simulink model "Cable_Wo_M_Inductance_Modelling_Study"  (R2024b)
settings: Solver=FixedStepDiscrete  StartTime=0.0  StopTime=5  FixedStep=1e-6  RelTol=1e-3  AbsTol=1
values from neighbouring files (symbols this model uses):
  Ccs1 = 733.62e-12    (= 7.3362e-10)    [Cable_Data_Inductance_Study.m]
  Ccs2 = 733.62e-12    (= 7.3362e-10)    [Cable_Data_Inductance_Study.m]
  Lc1 = 0.092e-6    (= 9.2e-08)    [Cable_Data_Inductance_Study.m]
  Lc1_total = Lc1 + Mcs1    (= 2.72e-07)    [Cable_Data_Inductance_Study.m]
  Lc2 = 0.092e-6    (= 9.2e-08)    [Cable_Data_Inductance_Study.m]
  Lc2_total = Lc2 + Mcs2    (= 2.72e-07)    [Cable_Data_Inductance_Study.m]
  Len35_batt1_HVJB1_neg = 0.600    (= 0.6)    [Cable_Data_Inductance_Study.m]
  Len35_batt1_HVJB1_pos = 0.750    (= 0.75)    [Cable_Data_Inductance_Study.m]
  Ls1_eff = Ls1 + Mss_cal    [Cable_Data_Inductance_Study.m]
  Ls2_eff = Ls2 + Mss_cal    [Cable_Data_Inductance_Study.m]
  Rc1 = 0.38e-3    (= 0.00038)    [Cable_Data_Inductance_Study.m]
  Rc2 = 0.38e-3    (= 0.00038)    [Cable_Data_Inductance_Study.m]
  Rs1 = 2.55e-3    (= 0.00255)    [Cable_Data_Inductance_Study.m]
  Rs2 = 2.55e-3    (= 0.00255)    [Cable_Data_Inductance_Study.m]
undefined symbols (not defined in the file or in its folder): DiscIntNeverNeededParam, Lns95, Lps95
libraries: spsSeriesRLCBranchLib x59, spsCurrentMeasurementLib x12, spsVoltageMeasurementLib x9, spsGroundLib x6, spsMultimeterLib x6, eeGeneralControl x2, spsVariableResistorLib x2, spsDCVoltageSourceLib x2, spspowerguiLib x1, sps_lib x1
(part 1 of 2)
settings Model: Creator=SUDHAK1  LastModifiedBy=SUDHAK1

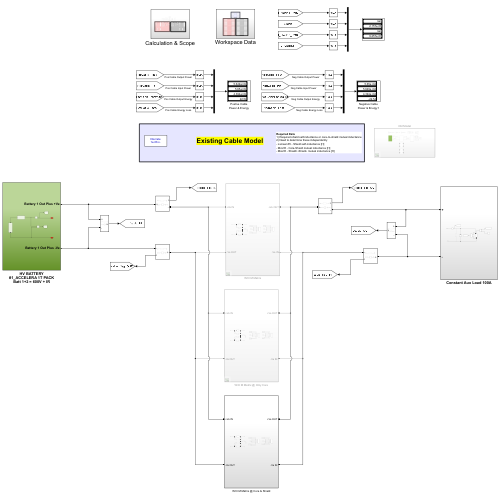
[thumbnail: Simulink's stored preview of the top-level diagram]
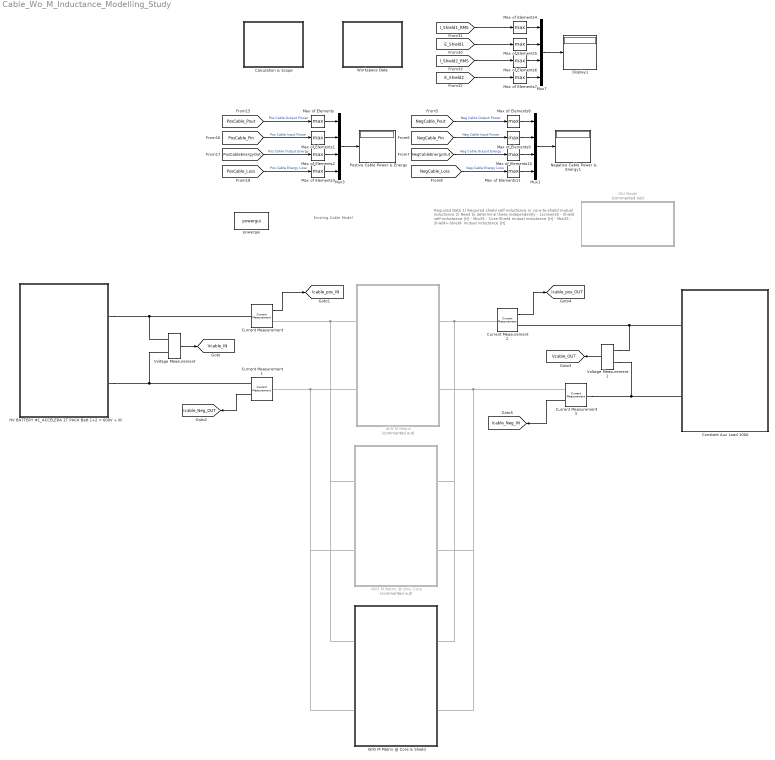
== system Cable_Wo_M_Inductance_Modelling_Study ==
  note: Required Data
      | 1) Required shield self-inductance or core-to-shield mutual inductance
      | 2) Need to determine these independently
      | - Lscreen35 - Shield self-inductance [H]
      | - Mcs35 - Core-Shield mutual inductance [H]
      | - Mss35 - Shield+-Shield- mutual inductance [H]
  note: Existing Cable Model
  Calculation & Scope : Subsystem
  Constant Aux Load 100A : Subsystem
  Current Measurement{,1..3} (4 alike) : spsCurrentMeasurementLib/Current Measurement  PhasorSimulation=off  OutputType=Complex  PSBequivalent=0
  Display1 : Display
  HV BATTERY #1_ACCELERA 1T PACK Batt 1+2 = 600V + IR : Subsystem
  Max of Elements{,1..11} (12 alike) : MinMax  Function=max
  Mux1 : Mux
  Mux3 : Mux
  Mux7 : Mux
  Negative Cable Power & Energy1 : Display
  Old Model : Subsystem  Commented=on
  Postive Cable Power & Energy : Display
  Voltage Measurement : spsVoltageMeasurementLib/Voltage Measurement  PhasorSimulation=off  OutputType=Complex  PSBequivalent=0
  Voltage Measurement1 : spsVoltageMeasurementLib/Voltage Measurement  PhasorSimulation=off  OutputType=Complex  PSBequivalent=0
  W/O M Matrix : Subsystem  Commented=on
  W/O M Matrix @ Core & Shield : Subsystem
  W/O M Matrix @ Only Core : Subsystem  Commented=on
  Workspace Data : Subsystem
  powergui : sps_lib/powergui  Priority=1  SimulationMode=Discrete  SampleTime=1e-6  frequency=60  Iterations=50  frequencyindice=0  Pbase=100e6  ErrMax=1e-4  UnitsV=kV  UnitsW=MW  buscounter=0  FunctionMessages=off  echomessages=off  EnableUseOfTLC=off  CurrentSourceSwitches=off  DisableSnubberDevices=off  DisableRonSwitches=off  DisableVfSwitches=off  DisplayEquations=off  AutomaticDiscreteSolvers=off  SolverType=Tustin/Backward Euler (TBE)  Interpol=off  ExternalGateDelay=off  methode=off  Ts=100  x0status=blocks  SPID=on  SwTol=0  HookPort=off  NonlinearTolerance=1e-4  nMaxIteration=100  ContinueOnMaxIteration=off  RestoreLinks=warning  ResistiveCurrentMeasurement=off  Frange=[0:2:500]  Ylog=off  Xlog=on  ShowGrid=off  save=off  variable=ZData  structure=0  ZoomFFT=off  StartTime=0.0  cycles=1  DisplayStyle=1  fundamental=60  FreqAxis=off  MaxFrequency=1000  frequencyindicesteady=1  RmsSteady=1  display=off
  tag scope: Icable_Neg_IN=global, Icable_Neg_OUT=global, Icable_pos_IN=global, Icable_pos_OUT=global, Vcable_IN=global, Vcable_OUT=global
  wires:
  Voltage Measurement1/1 -> [Vcable_OUT]
  Voltage Measurement/1 -> [Vcable_IN]
  Current Measurement/1 -> [Icable_pos_IN]
  Current Measurement3/1 -> [Icable_Neg_IN]
  Current Measurement1/1 -> [Icable_Neg_OUT]
  Current Measurement2/1 -> [Icable_pos_OUT]
  Max of Elements8/1 -> Mux1/1
  Mux1/1 -> Negative Cable Power & Energy1/1
  Max of Elements9/1 -> Mux1/2
  Max of Elements10/1 -> Mux1/3
  [PosCable_Pout] -> Max of Elements/1  "Pos Cable Output Power"
  Max of Elements11/1 -> Mux1/4
  [NegCableEnergyOut] -> Max of Elements10/1  "Neg Cable Output Energy"
  [PosCable_Pin] -> Max of Elements1/1  "Pos Cable Input Power"
  [E_Shield2] -> Max of Elements7/1
  Max of Elements7/1 -> Mux7/4
  Max of Elements5/1 -> Mux7/2
  [I_Shield2_RMS] -> Max of Elements6/1
  Max of Elements4/1 -> Mux7/1
  Max of Elements6/1 -> Mux7/3
  Mux7/1 -> Display1/1
  [E_Shield1] -> Max of Elements5/1
  [PosCableEnergyOut] -> Max of Elements2/1  "Pos Cable Output Energy"
  Max of Elements3/1 -> Mux3/4
  [I_Shield1_RMS] -> Max of Elements4/1
  [PosCable_Loss] -> Max of Elements3/1  "Pos Cable Energy Loss"
  Max of Elements2/1 -> Mux3/3
  [NegCable_Pin] -> Max of Elements9/1  "Neg Cable Input Power"
  Max of Elements/1 -> Mux3/1
  [NegCable_Loss] -> Max of Elements11/1  "Neg Cable Energy Loss"
  Max of Elements1/1 -> Mux3/2
  Mux3/1 -> Postive Cable Power & Energy/1
  [NegCable_Pout] -> Max of Elements8/1  "Neg Cable Output Power"
  connections:
  Voltage Measurement/LConn2 -- HV BATTERY #1_ACCELERA 1T PACK Batt 1+2 = 600V + IR/RConn2 -- Current Measurement1/RConn1
  Constant Aux Load 100A/RConn1 -- Voltage Measurement1/LConn1 -- Current Measurement2/RConn1
  Voltage Measurement1/LConn2 -- Constant Aux Load 100A/RConn2 -- Current Measurement3/LConn1
  HV BATTERY #1_ACCELERA 1T PACK Batt 1+2 = 600V + IR/RConn1 -- Voltage Measurement/LConn1 -- Current Measurement/LConn1
  W/O M Matrix/LConn1 -- W/O M Matrix @ Core & Shield/LConn1 -- W/O M Matrix @ Only Core/LConn1 -- Current Measurement/RConn1
  W/O M Matrix/RConn1 -- W/O M Matrix @ Core & Shield/RConn1 -- W/O M Matrix @ Only Core/RConn1 -- Current Measurement2/LConn1
  W/O M Matrix/LConn2 -- W/O M Matrix @ Core & Shield/LConn2 -- W/O M Matrix @ Only Core/LConn2 -- Current Measurement1/LConn1
  W/O M Matrix/RConn2 -- W/O M Matrix @ Core & Shield/RConn2 -- W/O M Matrix @ Only Core/RConn2 -- Current Measurement3/RConn1

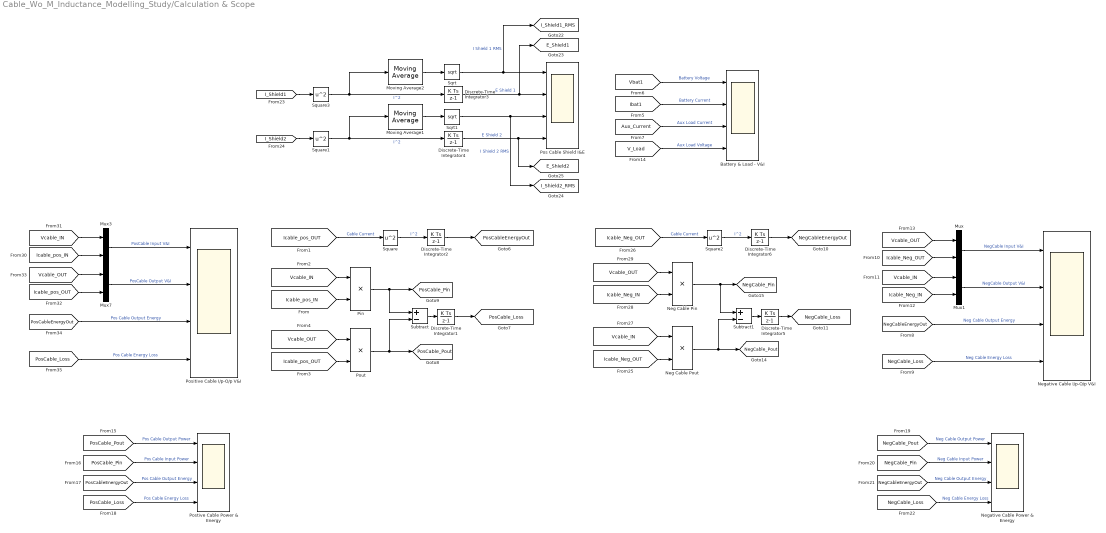
== system Cable_Wo_M_Inductance_Modelling_Study/Calculation & Scope ==
  Battery & Load - V&I : Scope  NumInputPorts=4
  Discrete-Time Integrator{1..6} (6 alike) : DiscreteIntegrator  SampleTime=-1  ICPrevOutput=DiscIntNeverNeededParam  ICPrevScaledInput=DiscIntNeverNeededParam
  Moving Average1 : eeGeneralControl/Moving Average  VariantControl=Variant1  LabelModeActiveChoice=Discrete  f=60  x0=0  BufferSize=8192  Ts=-1
  Moving Average2 : eeGeneralControl/Moving Average  VariantControl=Variant1  LabelModeActiveChoice=Discrete  f=60  x0=0  BufferSize=8192  Ts=-1
  Mux{,1,3,7} (4 alike) : Mux  Inputs=2
  Neg Cable Pin : Product
  Neg Cable Pout : Product
  Negative Cable Power & Energy : Scope  NumInputPorts=4
  Negative Cable I/p-O/p V&I : Scope  NumInputPorts=4
  Pin : Product
  Pos Cable Shield I&E : Scope  NumInputPorts=4
  Positive Cable I/p-O/p V&I : Scope  NumInputPorts=4
  Postive Cable Power & Energy : Scope  NumInputPorts=4
  Pout : Product
  Sqrt : Sqrt
  Sqrt1 : Sqrt
  Square{,1..3} (4 alike) : Math  Operator=square
  Subtract : Sum  Inputs=+-
  Subtract1 : Sum  Inputs=+-
  tag scope: E_Shield1=global, E_Shield2=global, I_Shield1_RMS=global, I_Shield2_RMS=global, NegCableEnergyOut=global, NegCable_Loss=global, NegCable_Pin=global, NegCable_Pout=global, PosCableEnergyOut=global, PosCable_Loss=global, PosCable_Pin=global, PosCable_Pout=global
  wires:
  [NegCableEnergyOut] -> Negative Cable I/p-O/p V&I/3  "Neg Cable Output Energy"
  Moving Average2/1 -> Sqrt/1
  Square/1 -> Discrete-Time Integrator2/1  "I^2"
  [Icable_pos_IN] -> Pin/2
  [PosCableEnergyOut] -> Postive Cable Power & Energy/3  "Pos Cable Output Energy"
  [Icable_pos_OUT] -> Pout/2
  [Icable_pos_OUT] -> Square/1  "Cable Current"
  Moving Average1/1 -> Sqrt1/1
  Discrete-Time Integrator3/1 -> [E_Shield1], Pos Cable Shield I&E/2  "E Shield 1"
  Pin/1 -> [PosCable_Pin], Subtract/1
  [Vcable_OUT] -> Pout/1
  Mux/1 -> Negative Cable I/p-O/p V&I/1  "NegCable Input V&I"
  [Aux_Current] -> Battery & Load - V&I/3  "Aux Load Current"
  [V_Load] -> Battery & Load - V&I/4  "Aux Load Voltage"
  [Icable_Neg_OUT] -> Mux/2
  Discrete-Time Integrator4/1 -> Pos Cable Shield I&E/4, [E_Shield2]  "E Shield 2"
  Square3/1 -> Discrete-Time Integrator3/1, Moving Average2/1  "I^2"
  [I_Shield1] -> Square3/1
  [Vbat1] -> Battery & Load - V&I/1  "Battery Voltage"
  Discrete-Time Integrator1/1 -> [PosCable_Loss]
  Sqrt1/1 -> Pos Cable Shield I&E/3, [I_Shield2_RMS]  "I Shield 2 RMS"
  [Vcable_IN] -> Neg Cable Pout/1
  [NegCable_Loss] -> Negative Cable I/p-O/p V&I/4  "Neg Cable Energy Loss"
  Subtract/1 -> Discrete-Time Integrator1/1
  Pout/1 -> Subtract/2, [PosCable_Pout]
  [Icable_Neg_OUT] -> Square2/1  "Cable Current"
  [PosCable_Pin] -> Postive Cable Power & Energy/2  "Pos Cable Input Power"
  [I_Shield2] -> Square1/1
  Mux1/1 -> Negative Cable I/p-O/p V&I/2  "NegCable Output V&I"
  Discrete-Time Integrator2/1 -> [PosCableEnergyOut]
  [Vcable_IN] -> Pin/1
  Square1/1 -> Discrete-Time Integrator4/1, Moving Average1/1  "I^2"
  [Icable_Neg_IN] -> Mux1/2
  [PosCable_Pout] -> Postive Cable Power & Energy/1  "Pos Cable Output Power"
  [PosCable_Loss] -> Postive Cable Power & Energy/4  "Pos Cable Energy Loss"
  [Ibat1] -> Battery & Load - V&I/2  "Battery Current"
  Sqrt/1 -> Pos Cable Shield I&E/1, [I_Shield1_RMS]  "I Shield 1 RMS"
  Subtract1/1 -> Discrete-Time Integrator5/1
  Discrete-Time Integrator5/1 -> [NegCable_Loss]
  Neg Cable Pout/1 -> Subtract1/2, [NegCable_Pout]
  Discrete-Time Integrator6/1 -> [NegCableEnergyOut]
  [Vcable_OUT] -> Neg Cable Pin/1
  Neg Cable Pin/1 -> Subtract1/1, [NegCable_Pin]
  [Icable_Neg_IN] -> Neg Cable Pin/2
  [Icable_Neg_OUT] -> Neg Cable Pout/2
  Square2/1 -> Discrete-Time Integrator6/1  "I^2"
  [NegCable_Loss] -> Negative Cable Power & Energy/4  "Neg Cable Energy Loss"
  [NegCableEnergyOut] -> Negative Cable Power & Energy/3  "Neg Cable Output Energy"
  [NegCable_Pout] -> Negative Cable Power & Energy/1  "Neg Cable Output Power"
  [NegCable_Pin] -> Negative Cable Power & Energy/2  "Neg Cable Input Power"
  [Icable_pos_IN] -> Mux3/2
  [Vcable_IN] -> Mux3/1
  [Icable_pos_OUT] -> Mux7/2
  [PosCable_Loss] -> Positive Cable I/p-O/p V&I/4  "Pos Cable Energy Loss"
  Mux3/1 -> Positive Cable I/p-O/p V&I/1  "PosCable Input V&I"
  Mux7/1 -> Positive Cable I/p-O/p V&I/2  "PosCable Output V&I"
  [Vcable_OUT] -> Mux7/1
  [PosCableEnergyOut] -> Positive Cable I/p-O/p V&I/3  "Pos Cable Output Energy"
  [Vcable_IN] -> Mux1/1
  [Vcable_OUT] -> Mux/1

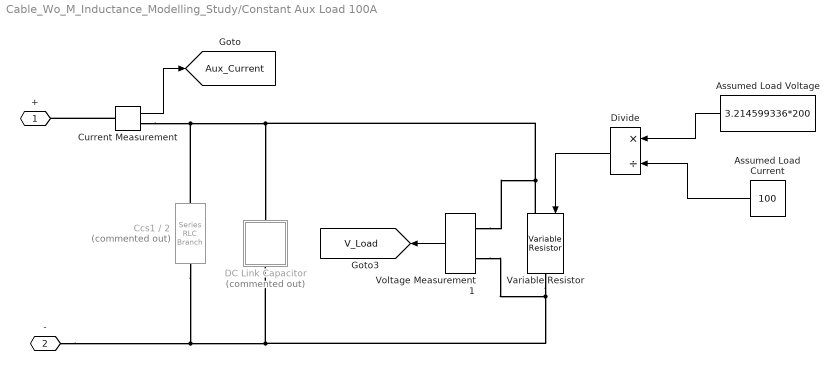
== system Cable_Wo_M_Inductance_Modelling_Study/Constant Aux Load 100A ==
  " Ccs1 / 2" : spsSeriesRLCBranchLib/Series RLC Branch  Commented=on  LConnTagsString=__new0  RConnTagsString=__new0  BranchType=R  Resistance=1  Inductance=1e-3  SetiL0=off  InitialCurrent=0  Capacitance=Ccs1/2  Setx0=off  InitialVoltage=0  Measurements=None
  Assumed Load Current : Constant  Value=100
  Assumed Load Voltage : Constant  Value=3.214599336*200
  Current Measurement : spsCurrentMeasurementLib/Current Measurement  PhasorSimulation=off  OutputType=Complex  PSBequivalent=0
  DC Link Capacitor : Subsystem  Commented=on
      settings: PortSchema="{\"entries\":[{\"content\":{\"sides\":[{\"content\":{},\"type\":\"ConnectorPlacement.EquallySpacedRectSide\",\"uuid\":\"a9c9044e-480e-49f2-9d9a-ad6fbdeb65df\"},{\"content\":{\"side\":\"RIGHT\"},\"type\":\"ConnectorPlacement.EquallySpacedRectSide\",\"uuid\":\"db4a4fc7-6a64-44bf-88d6-5d8062a8668f\"},{\"content\":{\"connectorIds\":[\"LConn1\"],\"side\":\"TOP\"},\"type\":\"ConnectorPlacement.EquallySpacedRectSide\",\"uuid\":\"c4fbeb8e-5c35-4874-aa8f-a5810cded374\"},{\"content\":{\"connectorIds\":[\"RConn1\"],\"side\":\"BOTTOM\"},\"type\":\"ConnectorPlacement.EquallySpacedRectSide\",\"uuid\":\"95f71b14-027a-489a-83bf-19494ef52344\"}]},\"type\":\"ConnectorPlacement.EquallySpacedConnector\",\"uuid\":\"3c0edebe-2bcc-4259-9d3a-139f17972178\"}],\"packageUris\":[\"http://schema.mathworks.com/mf0/Connector/R2020b\"],\"version\":\"1.0\"}"
  Divide : Product  Inputs=*/
  Variable Resistor : spsVariableResistorLib/Variable Resistor  Rabsmin=1e-3
  Voltage Measurement1 : spsVoltageMeasurementLib/Voltage Measurement  PhasorSimulation=off  OutputType=Complex  PSBequivalent=0
  + : PMIOPort  Side=Right
  - : PMIOPort  Port=2  Side=Right
  tag scope: Aux_Current=global, V_Load=global
  wires:
  Current Measurement/1 -> [Aux_Current]
  Divide/1 -> Variable Resistor/1
  Assumed Load Current/1 -> Divide/2
  Assumed Load Voltage/1 -> Divide/1
  Voltage Measurement1/1 -> [V_Load]
  connections:
  Current Measurement/LConn1 -- +/RConn1
  Current Measurement/RConn1 -- " Ccs1 / 2"/LConn1 -- Variable Resistor/LConn1 -- Voltage Measurement1/LConn1 -- DC Link Capacitor/RConn1
  -/RConn1 -- Voltage Measurement1/LConn2 -- Variable Resistor/RConn1 -- DC Link Capacitor/LConn1 -- " Ccs1 / 2"/RConn1

== system Cable_Wo_M_Inductance_Modelling_Study/HV BATTERY #1_ACCELERA 1T PACK Batt 1+2 = 600V + IR ==
  Battery-1 IR : spsSeriesRLCBranchLib/Series RLC Branch  LConnTagsString=__new0  RConnTagsString=__new0  BranchType=R  Resistance=(2.14417*200)*1e-3  Inductance=1e-3  SetiL0=off  InitialCurrent=0  Capacitance=1e-6  Setx0=off  InitialVoltage=0  Measurements=None
  Battery-1 OCV : spsDCVoltageSourceLib/DC Voltage Source  Amplitude=3.214599336*200  Measurements=None
  Current Measurement1 : spsCurrentMeasurementLib/Current Measurement  PhasorSimulation=off  OutputType=Complex  PSBequivalent=0
  Voltage Measurement2 : spsVoltageMeasurementLib/Voltage Measurement  PhasorSimulation=off  OutputType=Complex  PSBequivalent=0
  Battery 1 Out Plus +Ve : PMIOPort  Side=Right
  Battery 1 Out Plus -Ve : PMIOPort  Port=2  Side=Right
  tag scope: Ibat1=global, Vbat1=global
  wires:
  Voltage Measurement2/1 -> [Vbat1]
  Current Measurement1/1 -> [Ibat1]
  connections:
  Voltage Measurement2/LConn2 -- Battery-1 OCV/LConn1 -- Battery 1 Out Plus -Ve/RConn1
  Voltage Measurement2/LConn1 -- Current Measurement1/LConn1 -- Battery-1 IR/RConn1
  Current Measurement1/RConn1 -- Battery 1 Out Plus +Ve/RConn1
  Battery-1 OCV/RConn1 -- Battery-1 IR/LConn1

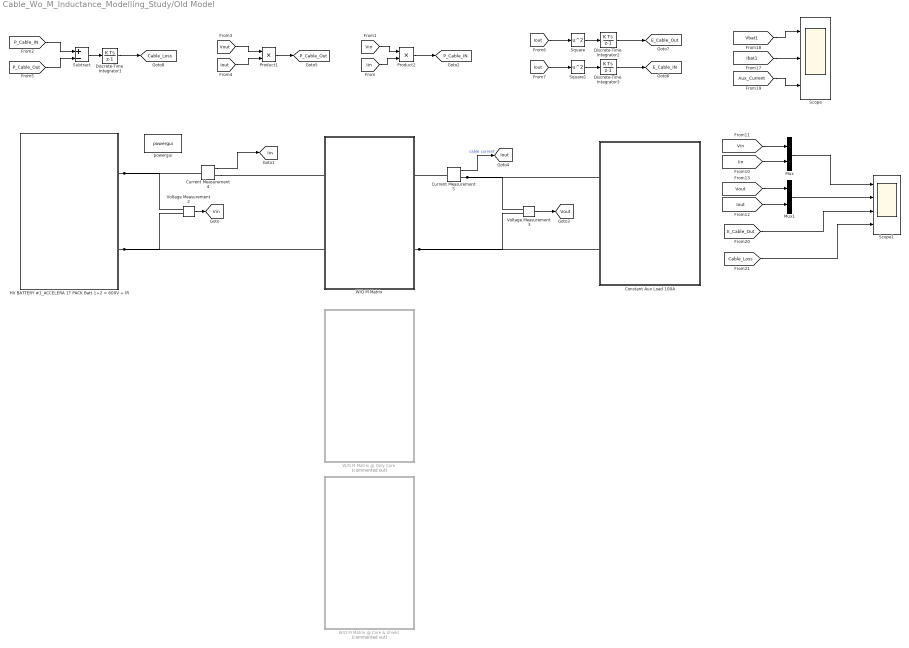
== system Cable_Wo_M_Inductance_Modelling_Study/Old Model ==
  Constant Aux Load 100A : Subsystem
  Current Measurement4 : spsCurrentMeasurementLib/Current Measurement  PhasorSimulation=off  OutputType=Complex  PSBequivalent=0
  Current Measurement5 : spsCurrentMeasurementLib/Current Measurement  PhasorSimulation=off  OutputType=Complex  PSBequivalent=0
  Discrete-Time Integrator1 : DiscreteIntegrator  SampleTime=-1  ICPrevOutput=DiscIntNeverNeededParam  ICPrevScaledInput=DiscIntNeverNeededParam
  Discrete-Time Integrator2 : DiscreteIntegrator  SampleTime=-1  ICPrevOutput=DiscIntNeverNeededParam  ICPrevScaledInput=DiscIntNeverNeededParam
  Discrete-Time Integrator3 : DiscreteIntegrator  SampleTime=-1  ICPrevOutput=DiscIntNeverNeededParam  ICPrevScaledInput=DiscIntNeverNeededParam
  HV BATTERY #1_ACCELERA 1T PACK Batt 1+2 = 600V + IR : Subsystem
  Mux : Mux  Inputs=2
  Mux1 : Mux  Inputs=2
  Product1 : Product
  Product2 : Product
  Scope : Scope  NumInputPorts=3
  Scope1 : Scope  NumInputPorts=4
  Square : Math  Operator=square
  Square1 : Math  Operator=square
  Subtract : Sum  Inputs=+-
  Voltage Measurement2 : spsVoltageMeasurementLib/Voltage Measurement  PhasorSimulation=off  OutputType=Complex  PSBequivalent=0
  Voltage Measurement3 : spsVoltageMeasurementLib/Voltage Measurement  PhasorSimulation=off  OutputType=Complex  PSBequivalent=0
  W/O M Matrix : Subsystem
  W/O M Matrix @ Core & Shield : Subsystem  Commented=on
  W/O M Matrix @ Only Core : Subsystem  Commented=on
  powergui : spspowerguiLib/powergui  Priority=1  SimulationMode=Discrete  SampleTime=1e-6  frequency=60  Iterations=50  frequencyindice=0  Pbase=100e6  ErrMax=1e-4  UnitsV=kV  UnitsW=MW  buscounter=0  FunctionMessages=off  echomessages=off  EnableUseOfTLC=off  CurrentSourceSwitches=off  DisableSnubberDevices=off  DisableRonSwitches=off  DisableVfSwitches=off  DisplayEquations=off  AutomaticDiscreteSolvers=off  SolverType=Tustin/Backward Euler (TBE)  Interpol=off  ExternalGateDelay=off  methode=off  Ts=100  x0status=blocks  SPID=on  SwTol=0  HookPort=off  NonlinearTolerance=1e-4  nMaxIteration=100  ContinueOnMaxIteration=off  RestoreLinks=warning  ResistiveCurrentMeasurement=off  Frange=[0:2:500]  Ylog=off  Xlog=on  ShowGrid=off  save=off  variable=ZData  structure=0  ZoomFFT=off  StartTime=0.0  cycles=1  DisplayStyle=1  fundamental=60  FreqAxis=off  MaxFrequency=1000  frequencyindicesteady=1  RmsSteady=1  display=off
  tag scope: Cable_Loss=global, E_Cable_IN=global, E_Cable_Out=global, Iin=global, Iout=global, P_Cable_IN=global, P_Cable_Out=global, Vin=global, Vout=global
  wires:
  Product2/1 -> [P_Cable_IN]
  [Aux_Current] -> Scope/3
  Voltage Measurement2/1 -> [Vin]
  [Iout] -> Mux1/2
  Square/1 -> Discrete-Time Integrator2/1
  Discrete-Time Integrator1/1 -> [Cable_Loss]
  [Vin] -> Product2/1
  [Iout] -> Product1/2
  Square1/1 -> Discrete-Time Integrator3/1
  Mux1/1 -> Scope1/2
  Voltage Measurement3/1 -> [Vout]
  Subtract/1 -> Discrete-Time Integrator1/1
  [Vout] -> Product1/1
  [Cable_Loss] -> Scope1/4
  [Iin] -> Product2/2
  [Vbat1] -> Scope/1
  Discrete-Time Integrator3/1 -> [E_Cable_IN]
  [Vout] -> Mux1/1
  [P_Cable_IN] -> Subtract/1
  [P_Cable_Out] -> Subtract/2
  [E_Cable_Out] -> Scope1/3
  [Iout] -> Square/1
  Current Measurement5/1 -> [Iout]  "cable current"
  [Ibat1] -> Scope/2
  [Iout] -> Square1/1
  Current Measurement4/1 -> [Iin]
  Discrete-Time Integrator2/1 -> [E_Cable_Out]
  Mux/1 -> Scope1/1
  [Vin] -> Mux/1
  [Iin] -> Mux/2
  Product1/1 -> [P_Cable_Out]
  connections:
  W/O M Matrix/RConn2 -- Voltage Measurement3/LConn2 -- Constant Aux Load 100A/RConn2
  Current Measurement4/RConn1 -- W/O M Matrix/LConn1
  Current Measurement5/LConn1 -- W/O M Matrix/RConn1
  Current Measurement5/RConn1 -- Voltage Measurement3/LConn1 -- Constant Aux Load 100A/RConn1
  HV BATTERY #1_ACCELERA 1T PACK Batt 1+2 = 600V + IR/RConn2 -- Voltage Measurement2/LConn2 -- W/O M Matrix/LConn2
  HV BATTERY #1_ACCELERA 1T PACK Batt 1+2 = 600V + IR/RConn1 -- Voltage Measurement2/LConn1 -- Current Measurement4/LConn1

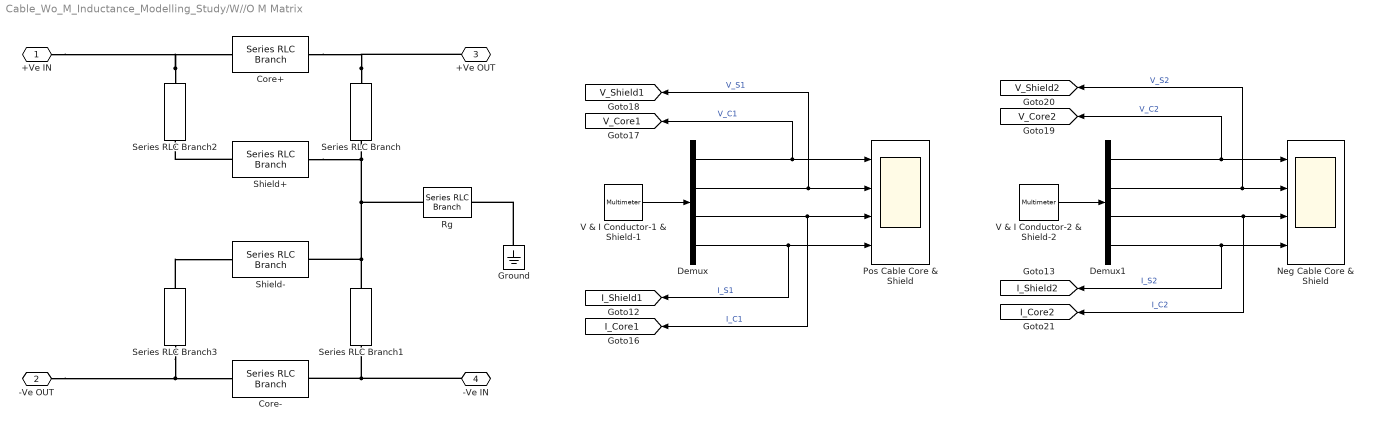
== system Cable_Wo_M_Inductance_Modelling_Study/W//O M Matrix ==
  Core+ : spsSeriesRLCBranchLib/Series RLC Branch  LConnTagsString=__new0  RConnTagsString=__new0  BranchType=RL  Resistance=Rc1*Len35_batt1_HVJB1_pos  Inductance=Lc1*Len35_batt1_HVJB1_pos  SetiL0=off  InitialCurrent=0  Capacitance=1e-6  Setx0=off  InitialVoltage=0  Measurements=Branch voltage and current
  Core- : spsSeriesRLCBranchLib/Series RLC Branch  LConnTagsString=__new0  RConnTagsString=__new0  BranchType=RL  Resistance=Rc2*Len35_batt1_HVJB1_neg  Inductance=Lc2*Len35_batt1_HVJB1_neg  SetiL0=off  InitialCurrent=0  Capacitance=1e-6  Setx0=off  InitialVoltage=0  Measurements=Branch voltage and current
  Demux : Demux
  Demux1 : Demux
  Ground : spsGroundLib/Ground  LConnTagsString=a
  Neg Cable Core & Shield : Scope  NumInputPorts=4
  Pos Cable Core & Shield : Scope  NumInputPorts=4
  Rg : spsSeriesRLCBranchLib/Series RLC Branch  LConnTagsString=__new0  RConnTagsString=__new0  BranchType=R  Resistance=10e-03  Inductance=1e-3  SetiL0=off  InitialCurrent=0  Capacitance=1e-6  Setx0=off  InitialVoltage=0  Measurements=Branch voltage and current
  Series RLC Branch : spsSeriesRLCBranchLib/Series RLC Branch  LConnTagsString=__new0  RConnTagsString=__new0  BranchType=C  Resistance=1  Inductance=1e-3  SetiL0=off  InitialCurrent=0  Capacitance=(Ccs1/2)*Len35_batt1_HVJB1_pos  Setx0=off  InitialVoltage=0  Measurements=None
  Series RLC Branch1 : spsSeriesRLCBranchLib/Series RLC Branch  LConnTagsString=__new0  RConnTagsString=__new0  BranchType=C  Resistance=1  Inductance=1e-3  SetiL0=off  InitialCurrent=0  Capacitance=(Ccs2/2)*Len35_batt1_HVJB1_neg  Setx0=off  InitialVoltage=0  Measurements=None
  Series RLC Branch2 : spsSeriesRLCBranchLib/Series RLC Branch  LConnTagsString=__new0  RConnTagsString=__new0  BranchType=C  Resistance=1  Inductance=1e-3  SetiL0=off  InitialCurrent=0  Capacitance=(Ccs1/2)*Len35_batt1_HVJB1_pos  Setx0=off  InitialVoltage=0  Measurements=None
  Series RLC Branch3 : spsSeriesRLCBranchLib/Series RLC Branch  LConnTagsString=__new0  RConnTagsString=__new0  BranchType=C  Resistance=1  Inductance=1e-3  SetiL0=off  InitialCurrent=0  Capacitance=(Ccs2/2)*Len35_batt1_HVJB1_neg  Setx0=off  InitialVoltage=0  Measurements=None
  Shield+ : spsSeriesRLCBranchLib/Series RLC Branch  LConnTagsString=__new0  RConnTagsString=__new0  BranchType=R  Resistance=Rs1*Len35_batt1_HVJB1_pos  Inductance=1  SetiL0=off  InitialCurrent=0  Capacitance=1e-6  Setx0=off  InitialVoltage=0  Measurements=Branch voltage and current
  Shield- : spsSeriesRLCBranchLib/Series RLC Branch  LConnTagsString=__new0  RConnTagsString=__new0  BranchType=R  Resistance=Rs2*Len35_batt1_HVJB1_neg  Inductance=Lns95*3.305  SetiL0=off  InitialCurrent=0  Capacitance=1e-6  Setx0=off  InitialVoltage=0  Measurements=Branch voltage and current
  V & I Conductor-1 & Shield-1 : spsMultimeterLib/Multimeter  L=10  sel=[1 4 6 9]  yselected={}  Gain=[1 1 1 1]  OutputType=Complex  PlotAtSimulationStop=off  PhasorSimulation=off
  V & I Conductor-2 & Shield-2 : spsMultimeterLib/Multimeter  L=10  sel=[2 5 7 10]  yselected={}  Gain=[1 1 1 1]  OutputType=Complex  PlotAtSimulationStop=off  PhasorSimulation=off
  +Ve IN : PMIOPort  Side=Left
  -Ve OUT : PMIOPort  Port=2  Side=Left
  +Ve OUT : PMIOPort  Port=3  Side=Right
  -Ve IN : PMIOPort  Port=4  Side=Right
  tag scope: I_Core1=global, I_Core2=global, I_Shield1=global, I_Shield2=global, V_Core1=global, V_Core2=global, V_Shield1=global, V_Shield2=global
  wires:
  V & I Conductor-1 & Shield-1/1 -> Demux/1
  Demux/3 -> [I_Core1], Pos Cable Core & Shield/3  "I_C1"
  Demux/2 -> Pos Cable Core & Shield/2, [V_Shield1]  "V_S1"
  Demux/4 -> [I_Shield1], Pos Cable Core & Shield/4  "I_S1"
  Demux/1 -> Pos Cable Core & Shield/1, [V_Core1]  "V_C1"
  Demux1/3 -> [I_Core2], Neg Cable Core & Shield/3  "I_C2"
  Demux1/4 -> [I_Shield2], Neg Cable Core & Shield/4  "I_S2"
  Demux1/1 -> [V_Core2], Neg Cable Core & Shield/1  "V_C2"
  Demux1/2 -> Neg Cable Core & Shield/2, [V_Shield2]  "V_S2"
  V & I Conductor-2 & Shield-2/1 -> Demux1/1
  connections:
  Series RLC Branch3/LConn1 -- -Ve OUT/RConn1 -- Core-/LConn1
  Ground/LConn1 -- Rg/RConn1
  Series RLC Branch2/LConn1 -- +Ve IN/RConn1 -- Core+/LConn1
  Series RLC Branch/LConn1 -- +Ve OUT/RConn1 -- Core+/RConn1
  Shield+/LConn1 -- Series RLC Branch2/RConn1
  -Ve IN/RConn1 -- Series RLC Branch1/LConn1 -- Core-/RConn1
  Series RLC Branch1/RConn1 -- Series RLC Branch/RConn1 -- Shield+/RConn1 -- Rg/LConn1 -- Shield-/RConn1
  Series RLC Branch3/RConn1 -- Shield-/LConn1

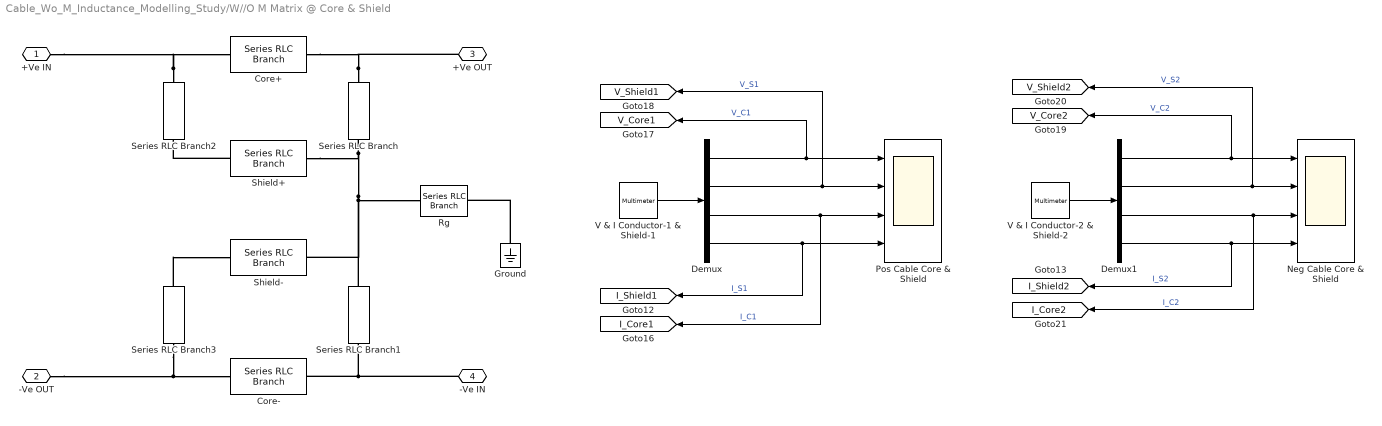
== system Cable_Wo_M_Inductance_Modelling_Study/W//O M Matrix @ Core & Shield ==
  Core+ : spsSeriesRLCBranchLib/Series RLC Branch  LConnTagsString=__new0  RConnTagsString=__new0  BranchType=RL  Resistance=Rc1*Len35_batt1_HVJB1_pos  Inductance=Lc1_total*Len35_batt1_HVJB1_pos  SetiL0=off  InitialCurrent=0  Capacitance=1e-6  Setx0=off  InitialVoltage=0  Measurements=Branch voltage and current
  Core- : spsSeriesRLCBranchLib/Series RLC Branch  LConnTagsString=__new0  RConnTagsString=__new0  BranchType=RL  Resistance=Rc2*Len35_batt1_HVJB1_neg  Inductance=Lc2_total*Len35_batt1_HVJB1_neg  SetiL0=off  InitialCurrent=0  Capacitance=1e-6  Setx0=off  InitialVoltage=0  Measurements=Branch voltage and current
  Demux : Demux
  Demux1 : Demux
  Ground : spsGroundLib/Ground  LConnTagsString=a
  Neg Cable Core & Shield : Scope  NumInputPorts=4
  Pos Cable Core & Shield : Scope  NumInputPorts=4
  Rg : spsSeriesRLCBranchLib/Series RLC Branch  LConnTagsString=__new0  RConnTagsString=__new0  BranchType=R  Resistance=10e-03  Inductance=1e-3  SetiL0=off  InitialCurrent=0  Capacitance=1e-6  Setx0=off  InitialVoltage=0  Measurements=Branch voltage and current
  Series RLC Branch : spsSeriesRLCBranchLib/Series RLC Branch  LConnTagsString=__new0  RConnTagsString=__new0  BranchType=C  Resistance=1  Inductance=1e-3  SetiL0=off  InitialCurrent=0  Capacitance=(Ccs1/2)*Len35_batt1_HVJB1_pos  Setx0=off  InitialVoltage=0  Measurements=None
  Series RLC Branch1 : spsSeriesRLCBranchLib/Series RLC Branch  LConnTagsString=__new0  RConnTagsString=__new0  BranchType=C  Resistance=1  Inductance=1e-3  SetiL0=off  InitialCurrent=0  Capacitance=(Ccs2/2)*Len35_batt1_HVJB1_neg  Setx0=off  InitialVoltage=0  Measurements=None
  Series RLC Branch2 : spsSeriesRLCBranchLib/Series RLC Branch  LConnTagsString=__new0  RConnTagsString=__new0  BranchType=C  Resistance=1  Inductance=1e-3  SetiL0=off  InitialCurrent=0  Capacitance=(Ccs1/2)*Len35_batt1_HVJB1_pos  Setx0=off  InitialVoltage=0  Measurements=None
  Series RLC Branch3 : spsSeriesRLCBranchLib/Series RLC Branch  LConnTagsString=__new0  RConnTagsString=__new0  BranchType=C  Resistance=1  Inductance=1e-3  SetiL0=off  InitialCurrent=0  Capacitance=(Ccs2/2)*Len35_batt1_HVJB1_neg  Setx0=off  InitialVoltage=0  Measurements=None
  Shield+ : spsSeriesRLCBranchLib/Series RLC Branch  LConnTagsString=__new0  RConnTagsString=__new0  BranchType=RL  Resistance=Rs1*Len35_batt1_HVJB1_pos  Inductance=Ls1_eff*Len35_batt1_HVJB1_pos  SetiL0=off  InitialCurrent=0  Capacitance=1e-6  Setx0=off  InitialVoltage=0  Measurements=Branch voltage and current
  Shield- : spsSeriesRLCBranchLib/Series RLC Branch  LConnTagsString=__new0  RConnTagsString=__new0  BranchType=RL  Resistance=Rs2*Len35_batt1_HVJB1_neg  Inductance=Ls2_eff*Len35_batt1_HVJB1_neg  SetiL0=off  InitialCurrent=0  Capacitance=1e-6  Setx0=off  InitialVoltage=0  Measurements=Branch voltage and current
  V & I Conductor-1 & Shield-1 : spsMultimeterLib/Multimeter  L=10  sel=[1 4 6 9]  yselected={}  Gain=[1 1 1 1]  OutputType=Complex  PlotAtSimulationStop=off  PhasorSimulation=off
  V & I Conductor-2 & Shield-2 : spsMultimeterLib/Multimeter  L=10  sel=[2 5 7 10]  yselected={}  Gain=[1 1 1 1]  OutputType=Complex  PlotAtSimulationStop=off  PhasorSimulation=off
  +Ve IN : PMIOPort  Side=Left
  -Ve OUT : PMIOPort  Port=2  Side=Left
  +Ve OUT : PMIOPort  Port=3  Side=Right
  -Ve IN : PMIOPort  Port=4  Side=Right
  tag scope: I_Core1=global, I_Core2=global, I_Shield1=global, I_Shield2=global, V_Core1=global, V_Core2=global, V_Shield1=global, V_Shield2=global
  wires:
  Demux1/1 -> [V_Core2], Neg Cable Core & Shield/1  "V_C2"
  V & I Conductor-2 & Shield-2/1 -> Demux1/1
  Demux/1 -> Pos Cable Core & Shield/1, [V_Core1]  "V_C1"
  Demux/2 -> Pos Cable Core & Shield/2, [V_Shield1]  "V_S1"
  Demux/4 -> [I_Shield1], Pos Cable Core & Shield/4  "I_S1"
  Demux1/2 -> Neg Cable Core & Shield/2, [V_Shield2]  "V_S2"
  V & I Conductor-1 & Shield-1/1 -> Demux/1
  Demux/3 -> [I_Core1], Pos Cable Core & Shield/3  "I_C1"
  Demux1/4 -> [I_Shield2], Neg Cable Core & Shield/4  "I_S2"
  Demux1/3 -> [I_Core2], Neg Cable Core & Shield/3  "I_C2"
  connections:
  Series RLC Branch3/LConn1 -- -Ve OUT/RConn1 -- Core-/LConn1
  Ground/LConn1 -- Rg/RConn1
  Series RLC Branch2/LConn1 -- +Ve IN/RConn1 -- Core+/LConn1
  Series RLC Branch/LConn1 -- +Ve OUT/RConn1 -- Core+/RConn1
  Series RLC Branch/RConn1 -- Shield+/RConn1 -- Series RLC Branch1/RConn1 -- Shield-/RConn1 -- Rg/LConn1
  -Ve IN/RConn1 -- Series RLC Branch1/LConn1 -- Core-/RConn1
  Series RLC Branch3/RConn1 -- Shield-/LConn1
  Shield+/LConn1 -- Series RLC Branch2/RConn1

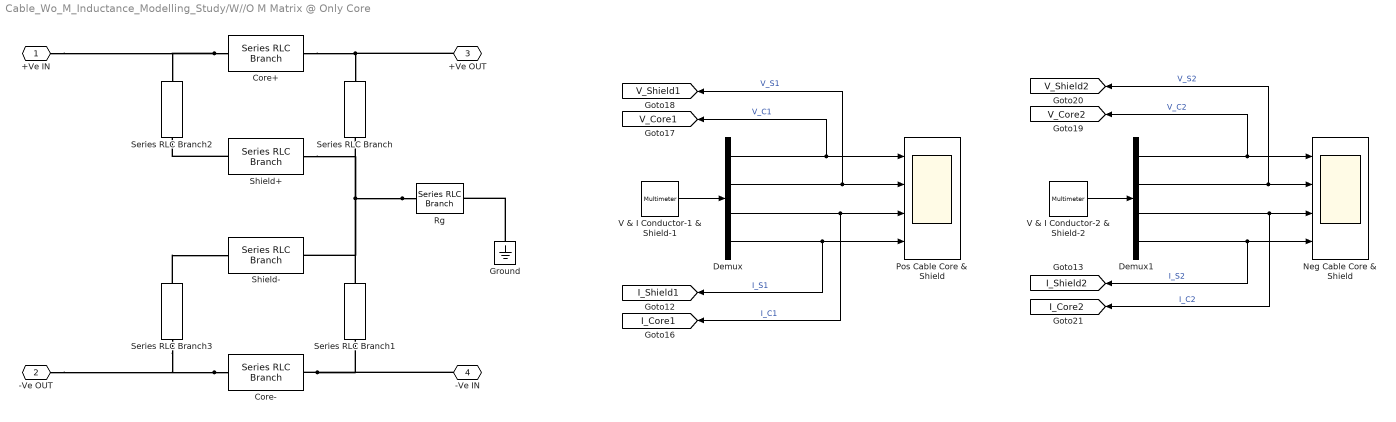
== system Cable_Wo_M_Inductance_Modelling_Study/W//O M Matrix @ Only Core ==
  Core+ : spsSeriesRLCBranchLib/Series RLC Branch  LConnTagsString=__new0  RConnTagsString=__new0  BranchType=RL  Resistance=Rc1*Len35_batt1_HVJB1_pos  Inductance=Lc1_total*Len35_batt1_HVJB1_pos  SetiL0=off  InitialCurrent=0  Capacitance=1e-6  Setx0=off  InitialVoltage=0  Measurements=Branch voltage and current
  Core- : spsSeriesRLCBranchLib/Series RLC Branch  LConnTagsString=__new0  RConnTagsString=__new0  BranchType=RL  Resistance=Rc2*Len35_batt1_HVJB1_neg  Inductance=Lc2_total*Len35_batt1_HVJB1_neg  SetiL0=off  InitialCurrent=0  Capacitance=1e-6  Setx0=off  InitialVoltage=0  Measurements=Branch voltage and current
  Demux : Demux
  Demux1 : Demux
  Ground : spsGroundLib/Ground  LConnTagsString=a
  Neg Cable Core & Shield : Scope  NumInputPorts=4
  Pos Cable Core & Shield : Scope  NumInputPorts=4
  Rg : spsSeriesRLCBranchLib/Series RLC Branch  LConnTagsString=__new0  RConnTagsString=__new0  BranchType=R  Resistance=10e-03  Inductance=1e-3  SetiL0=off  InitialCurrent=0  Capacitance=1e-6  Setx0=off  InitialVoltage=0  Measurements=Branch voltage and current
  Series RLC Branch : spsSeriesRLCBranchLib/Series RLC Branch  LConnTagsString=__new0  RConnTagsString=__new0  BranchType=C  Resistance=1  Inductance=1e-3  SetiL0=off  InitialCurrent=0  Capacitance=(Ccs1/2)*Len35_batt1_HVJB1_pos  Setx0=off  InitialVoltage=0  Measurements=None
  Series RLC Branch1 : spsSeriesRLCBranchLib/Series RLC Branch  LConnTagsString=__new0  RConnTagsString=__new0  BranchType=C  Resistance=1  Inductance=1e-3  SetiL0=off  InitialCurrent=0  Capacitance=(Ccs2/2)*Len35_batt1_HVJB1_neg  Setx0=off  InitialVoltage=0  Measurements=None
  Series RLC Branch2 : spsSeriesRLCBranchLib/Series RLC Branch  LConnTagsString=__new0  RConnTagsString=__new0  BranchType=C  Resistance=1  Inductance=1e-3  SetiL0=off  InitialCurrent=0  Capacitance=(Ccs1/2)*Len35_batt1_HVJB1_pos  Setx0=off  InitialVoltage=0  Measurements=None
  Series RLC Branch3 : spsSeriesRLCBranchLib/Series RLC Branch  LConnTagsString=__new0  RConnTagsString=__new0  BranchType=C  Resistance=1  Inductance=1e-3  SetiL0=off  InitialCurrent=0  Capacitance=(Ccs2/2)*Len35_batt1_HVJB1_neg  Setx0=off  InitialVoltage=0  Measurements=None
  Shield+ : spsSeriesRLCBranchLib/Series RLC Branch  LConnTagsString=__new0  RConnTagsString=__new0  BranchType=R  Resistance=Rs1*Len35_batt1_HVJB1_pos  Inductance=Lps95*3.270  SetiL0=off  InitialCurrent=0  Capacitance=1e-6  Setx0=off  InitialVoltage=0  Measurements=Branch voltage and current
  Shield- : spsSeriesRLCBranchLib/Series RLC Branch  LConnTagsString=__new0  RConnTagsString=__new0  BranchType=R  Resistance=Rs2*Len35_batt1_HVJB1_neg  Inductance=Lns95*3.305  SetiL0=off  InitialCurrent=0  Capacitance=1e-6  Setx0=off  InitialVoltage=0  Measurements=Branch voltage and current
  V & I Conductor-1 & Shield-1 : spsMultimeterLib/Multimeter  L=10  sel=[1 4 6 9]  yselected={}  Gain=[1 1 1 1]  OutputType=Complex  PlotAtSimulationStop=off  PhasorSimulation=off
  V & I Conductor-2 & Shield-2 : spsMultimeterLib/Multimeter  L=10  sel=[2 5 7 10]  yselected={}  Gain=[1 1 1 1]  OutputType=Complex  PlotAtSimulationStop=off  PhasorSimulation=off
  +Ve IN : PMIOPort  Side=Left
  -Ve OUT : PMIOPort  Port=2  Side=Left
  +Ve OUT : PMIOPort  Port=3  Side=Right
  -Ve IN : PMIOPort  Port=4  Side=Right
  tag scope: I_Core1=global, I_Core2=global, I_Shield1=global, I_Shield2=global, V_Core1=global, V_Core2=global, V_Shield1=global, V_Shield2=global
  wires:
  Demux/4 -> [I_Shield1], Pos Cable Core & Shield/4  "I_S1"
  Demux/2 -> Pos Cable Core & Shield/2, [V_Shield1]  "V_S1"
  Demux/1 -> Pos Cable Core & Shield/1, [V_Core1]  "V_C1"
  Demux1/2 -> Neg Cable Core & Shield/2, [V_Shield2]  "V_S2"
  V & I Conductor-2 & Shield-2/1 -> Demux1/1
  Demux1/1 -> [V_Core2], Neg Cable Core & Shield/1  "V_C2"
  Demux1/4 -> [I_Shield2], Neg Cable Core & Shield/4  "I_S2"
  Demux/3 -> [I_Core1], Pos Cable Core & Shield/3  "I_C1"
  V & I Conductor-1 & Shield-1/1 -> Demux/1
  Demux1/3 -> [I_Core2], Neg Cable Core & Shield/3  "I_C2"
  connections:
  Core-/RConn1 -- Series RLC Branch1/LConn1 -- -Ve IN/RConn1
  Rg/LConn1 -- Shield-/RConn1 -- Series RLC Branch1/RConn1 -- Shield+/RConn1 -- Series RLC Branch/RConn1
  Core+/RConn1 -- +Ve OUT/RConn1 -- Series RLC Branch/LConn1
  Core+/LConn1 -- +Ve IN/RConn1 -- Series RLC Branch2/LConn1
  Ground/LConn1 -- Rg/RConn1
  Core-/LConn1 -- -Ve OUT/RConn1 -- Series RLC Branch3/LConn1
  Shield+/LConn1 -- Series RLC Branch2/RConn1
  Series RLC Branch3/RConn1 -- Shield-/LConn1

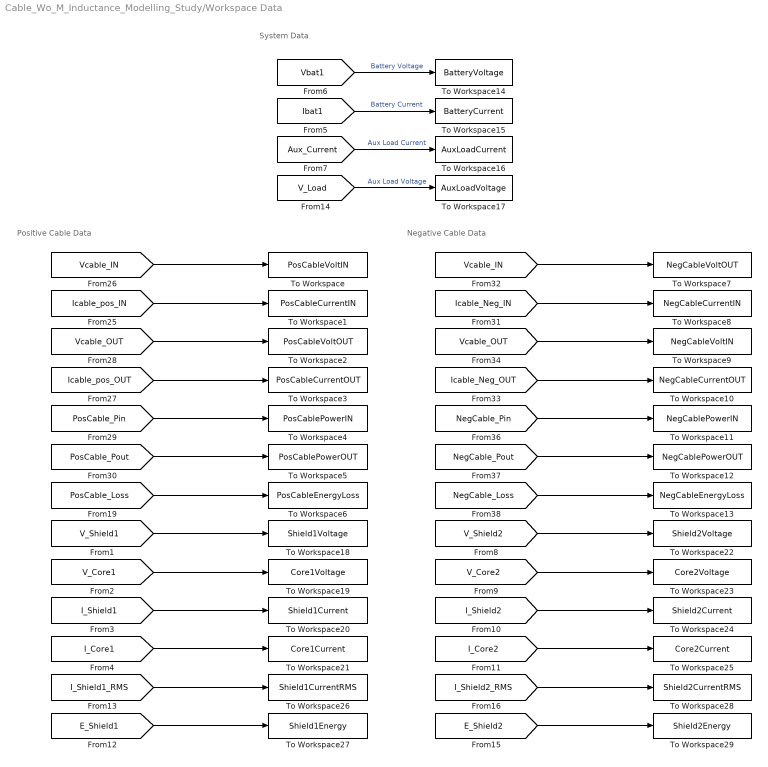
== system Cable_Wo_M_Inductance_Modelling_Study/Workspace Data ==
  note: System Data
  note: Negative Cable Data
  note: Positive Cable Data
  To Workspace : ToWorkspace  VariableName=PosCableVoltIN  SaveFormat=Timeseries  SampleTime=-1
  To Workspace1 : ToWorkspace  VariableName=PosCableCurrentIN  SaveFormat=Timeseries  SampleTime=-1
  To Workspace10 : ToWorkspace  VariableName=NegCableCurrentOUT  SaveFormat=Timeseries  SampleTime=-1
  To Workspace11 : ToWorkspace  VariableName=NegCablePowerIN  SaveFormat=Timeseries  SampleTime=-1
  To Workspace12 : ToWorkspace  VariableName=NegCablePowerOUT  SaveFormat=Timeseries  SampleTime=-1
  To Workspace13 : ToWorkspace  VariableName=NegCableEnergyLoss  SaveFormat=Timeseries  SampleTime=-1
  To Workspace14 : ToWorkspace  VariableName=BatteryVoltage  SaveFormat=Timeseries  SampleTime=-1
  To Workspace15 : ToWorkspace  VariableName=BatteryCurrent  SaveFormat=Timeseries  SampleTime=-1
  To Workspace16 : ToWorkspace  VariableName=AuxLoadCurrent  SaveFormat=Timeseries  SampleTime=-1
  To Workspace17 : ToWorkspace  VariableName=AuxLoadVoltage  SaveFormat=Timeseries  SampleTime=-1
  To Workspace18 : ToWorkspace  VariableName=Shield1Voltage  SaveFormat=Timeseries  SampleTime=-1
  To Workspace19 : ToWorkspace  VariableName=Core1Voltage  SaveFormat=Timeseries  SampleTime=-1
  To Workspace2 : ToWorkspace  VariableName=PosCableVoltOUT  SaveFormat=Timeseries  SampleTime=-1
  To Workspace20 : ToWorkspace  VariableName=Shield1Current  SaveFormat=Timeseries  SampleTime=-1
  To Workspace21 : ToWorkspace  VariableName=Core1Current  SaveFormat=Timeseries  SampleTime=-1
  To Workspace22 : ToWorkspace  VariableName=Shield2Voltage  SaveFormat=Timeseries  SampleTime=-1
  To Workspace23 : ToWorkspace  VariableName=Core2Voltage  SaveFormat=Timeseries  SampleTime=-1
  To Workspace24 : ToWorkspace  VariableName=Shield2Current  SaveFormat=Timeseries  SampleTime=-1
  To Workspace25 : ToWorkspace  VariableName=Core2Current  SaveFormat=Timeseries  SampleTime=-1
  To Workspace26 : ToWorkspace  VariableName=Shield1CurrentRMS  SaveFormat=Timeseries  SampleTime=-1
  To Workspace27 : ToWorkspace  VariableName=Shield1Energy  SaveFormat=Timeseries  SampleTime=-1
  To Workspace28 : ToWorkspace  VariableName=Shield2CurrentRMS  SaveFormat=Timeseries  SampleTime=-1
  To Workspace29 : ToWorkspace  VariableName=Shield2Energy  SaveFormat=Timeseries  SampleTime=-1
  To Workspace3 : ToWorkspace  VariableName=PosCableCurrentOUT  SaveFormat=Timeseries  SampleTime=-1
  To Workspace4 : ToWorkspace  VariableName=PosCablePowerIN  SaveFormat=Timeseries  SampleTime=-1
  To Workspace5 : ToWorkspace  VariableName=PosCablePowerOUT  SaveFormat=Timeseries  SampleTime=-1
  To Workspace6 : ToWorkspace  VariableName=PosCableEnergyLoss  SaveFormat=Timeseries  SampleTime=-1
  To Workspace7 : ToWorkspace  VariableName=NegCableVoltOUT  SaveFormat=Timeseries  SampleTime=-1
  To Workspace8 : ToWorkspace  VariableName=NegCableCurrentIN  SaveFormat=Timeseries  SampleTime=-1
  To Workspace9 : ToWorkspace  VariableName=NegCableVoltIN  SaveFormat=Timeseries  SampleTime=-1
  wires:
  [Ibat1] -> To Workspace15/1  "Battery Current"
  [Vbat1] -> To Workspace14/1  "Battery Voltage"
  [V_Load] -> To Workspace17/1  "Aux Load Voltage"
  [Aux_Current] -> To Workspace16/1  "Aux Load Current"
  [Vcable_IN] -> To Workspace/1
  [Icable_pos_IN] -> To Workspace1/1
  [Vcable_OUT] -> To Workspace2/1
  [Icable_pos_OUT] -> To Workspace3/1
  [PosCable_Pin] -> To Workspace4/1
  [PosCable_Pout] -> To Workspace5/1
  [PosCable_Loss] -> To Workspace6/1
  [NegCable_Loss] -> To Workspace13/1
  [NegCable_Pin] -> To Workspace11/1
  [Vcable_IN] -> To Workspace7/1
  [Vcable_OUT] -> To Workspace9/1
  [Icable_Neg_IN] -> To Workspace8/1
  [NegCable_Pout] -> To Workspace12/1
  [Icable_Neg_OUT] -> To Workspace10/1
  [V_Shield1] -> To Workspace18/1
  [V_Core1] -> To Workspace19/1
  [I_Shield1] -> To Workspace20/1
  [I_Core1] -> To Workspace21/1
  [V_Shield2] -> To Workspace22/1
  [V_Core2] -> To Workspace23/1
  [I_Shield2] -> To Workspace24/1
  [I_Core2] -> To Workspace25/1
  [I_Shield2_RMS] -> To Workspace28/1
  [E_Shield1] -> To Workspace27/1
  [I_Shield1_RMS] -> To Workspace26/1
  [E_Shield2] -> To Workspace29/1

== system Cable_Wo_M_Inductance_Modelling_Study/Constant Aux Load 100A/DC Link Capacitor ==
  Current Measurement1 : spsCurrentMeasurementLib/Current Measurement  PhasorSimulation=off  OutputType=Complex  PSBequivalent=0
  Cx : spsSeriesRLCBranchLib/Series RLC Branch  LConnTagsString=__new0  RConnTagsString=__new0  BranchType=C  Resistance=0.5  Inductance=1e-3  SetiL0=off  InitialCurrent=0  Capacitance=2e-3  Setx0=on  InitialVoltage=Cx_Vs  Measurements=Branch voltage and current
  To Workspace1 : ToWorkspace  VariableName=DCLinkCapVoltage  SaveFormat=Timeseries  SampleTime=-1
  To Workspace2 : ToWorkspace  VariableName=DCLinkCapCurrent  SaveFormat=Timeseries  SampleTime=-1
  Voltage Measurement : spsVoltageMeasurementLib/Voltage Measurement  PhasorSimulation=off  OutputType=Complex  PSBequivalent=0
  + : PMIOPort  Side=Left
  - : PMIOPort  Port=2  Side=Right
  wires:
  Voltage Measurement/1 -> To Workspace1/1
  Current Measurement1/1 -> To Workspace2/1
  connections:
  Current Measurement1/RConn1 -- -/RConn1 -- Voltage Measurement/LConn2
  Cx/RConn1 -- Current Measurement1/LConn1
  Voltage Measurement/LConn1 -- +/RConn1 -- Cx/LConn1

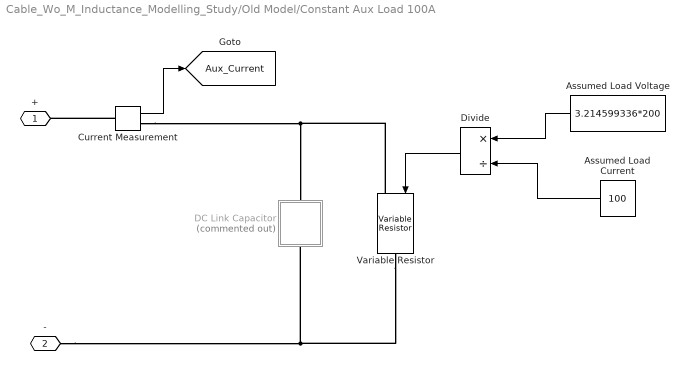
== system Cable_Wo_M_Inductance_Modelling_Study/Old Model/Constant Aux Load 100A ==
  Assumed Load Current : Constant  Value=100
  Assumed Load Voltage : Constant  Value=3.214599336*200
  Current Measurement : spsCurrentMeasurementLib/Current Measurement  PhasorSimulation=off  OutputType=Complex  PSBequivalent=0
  DC Link Capacitor : Subsystem  Commented=on
      settings: PortSchema="{\"entries\":[{\"content\":{\"sides\":[{\"content\":{},\"type\":\"ConnectorPlacement.EquallySpacedRectSide\",\"uuid\":\"a9c9044e-480e-49f2-9d9a-ad6fbdeb65df\"},{\"content\":{\"side\":\"RIGHT\"},\"type\":\"ConnectorPlacement.EquallySpacedRectSide\",\"uuid\":\"db4a4fc7-6a64-44bf-88d6-5d8062a8668f\"},{\"content\":{\"connectorIds\":[\"LConn1\"],\"side\":\"TOP\"},\"type\":\"ConnectorPlacement.EquallySpacedRectSide\",\"uuid\":\"c4fbeb8e-5c35-4874-aa8f-a5810cded374\"},{\"content\":{\"connectorIds\":[\"RConn1\"],\"side\":\"BOTTOM\"},\"type\":\"ConnectorPlacement.EquallySpacedRectSide\",\"uuid\":\"95f71b14-027a-489a-83bf-19494ef52344\"}]},\"type\":\"ConnectorPlacement.EquallySpacedConnector\",\"uuid\":\"3c0edebe-2bcc-4259-9d3a-139f17972178\"}],\"packageUris\":[\"http://schema.mathworks.com/mf0/Connector/R2020b\"],\"version\":\"1.0\"}"
  Divide : Product  Inputs=*/
  Variable Resistor : spsVariableResistorLib/Variable Resistor  Rabsmin=1e-3
  + : PMIOPort  Side=Right
  - : PMIOPort  Port=2  Side=Right
  tag scope: Aux_Current=global
  wires:
  Current Measurement/1 -> [Aux_Current]
  Divide/1 -> Variable Resistor/1
  Assumed Load Current/1 -> Divide/2
  Assumed Load Voltage/1 -> Divide/1
  connections:
  Current Measurement/LConn1 -- +/RConn1
  Current Measurement/RConn1 -- Variable Resistor/LConn1 -- DC Link Capacitor/RConn1
  -/RConn1 -- Variable Resistor/RConn1 -- DC Link Capacitor/LConn1

== system Cable_Wo_M_Inductance_Modelling_Study/Old Model/HV BATTERY #1_ACCELERA 1T PACK Batt 1+2 = 600V + IR ==
  Battery-1 IR : spsSeriesRLCBranchLib/Series RLC Branch  LConnTagsString=__new0  RConnTagsString=__new0  BranchType=R  Resistance=(2.14417*200)*1e-3  Inductance=1e-3  SetiL0=off  InitialCurrent=0  Capacitance=1e-6  Setx0=off  InitialVoltage=0  Measurements=None
  Battery-1 OCV : spsDCVoltageSourceLib/DC Voltage Source  Amplitude=3.214599336*200  Measurements=None
  Current Measurement1 : spsCurrentMeasurementLib/Current Measurement  PhasorSimulation=off  OutputType=Complex  PSBequivalent=0
  Voltage Measurement2 : spsVoltageMeasurementLib/Voltage Measurement  PhasorSimulation=off  OutputType=Complex  PSBequivalent=0
  Battery 1 Out Plus +Ve : PMIOPort  Side=Right
  Battery 1 Out Plus -Ve : PMIOPort  Port=2  Side=Right
  tag scope: Ibat1=global, Vbat1=global
  wires:
  Voltage Measurement2/1 -> [Vbat1]
  Current Measurement1/1 -> [Ibat1]
  connections:
  Voltage Measurement2/LConn2 -- Battery-1 OCV/LConn1 -- Battery 1 Out Plus -Ve/RConn1
  Voltage Measurement2/LConn1 -- Current Measurement1/LConn1 -- Battery-1 IR/RConn1
  Current Measurement1/RConn1 -- Battery 1 Out Plus +Ve/RConn1
  Battery-1 OCV/RConn1 -- Battery-1 IR/LConn1

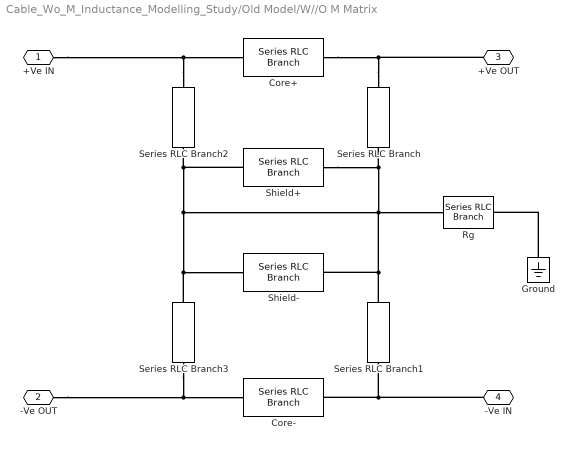
== system Cable_Wo_M_Inductance_Modelling_Study/Old Model/W//O M Matrix ==
  Core+ : spsSeriesRLCBranchLib/Series RLC Branch  LConnTagsString=__new0  RConnTagsString=__new0  BranchType=RL  Resistance=Rc1*Len35_batt1_HVJB1_pos  Inductance=Lc1*Len35_batt1_HVJB1_pos  SetiL0=off  InitialCurrent=0  Capacitance=1e-6  Setx0=off  InitialVoltage=0  Measurements=Branch voltage and current
  Core- : spsSeriesRLCBranchLib/Series RLC Branch  LConnTagsString=__new0  RConnTagsString=__new0  BranchType=RL  Resistance=Rc2*Len35_batt1_HVJB1_neg  Inductance=Lc2*Len35_batt1_HVJB1_neg  SetiL0=off  InitialCurrent=0  Capacitance=1e-6  Setx0=off  InitialVoltage=0  Measurements=Branch voltage and current
  Ground : spsGroundLib/Ground  LConnTagsString=a
  Rg : spsSeriesRLCBranchLib/Series RLC Branch  LConnTagsString=__new0  RConnTagsString=__new0  BranchType=R  Resistance=10e-03  Inductance=1e-3  SetiL0=off  InitialCurrent=0  Capacitance=1e-6  Setx0=off  InitialVoltage=0  Measurements=Branch voltage and current
  Series RLC Branch : spsSeriesRLCBranchLib/Series RLC Branch  LConnTagsString=__new0  RConnTagsString=__new0  BranchType=C  Resistance=1  Inductance=1e-3  SetiL0=off  InitialCurrent=0  Capacitance=(Ccs1/2)*Len35_batt1_HVJB1_pos  Setx0=off  InitialVoltage=0  Measurements=None
  Series RLC Branch1 : spsSeriesRLCBranchLib/Series RLC Branch  LConnTagsString=__new0  RConnTagsString=__new0  BranchType=C  Resistance=1  Inductance=1e-3  SetiL0=off  InitialCurrent=0  Capacitance=(Ccs2/2)*Len35_batt1_HVJB1_neg  Setx0=off  InitialVoltage=0  Measurements=None
  Series RLC Branch2 : spsSeriesRLCBranchLib/Series RLC Branch  LConnTagsString=__new0  RConnTagsString=__new0  BranchType=C  Resistance=1  Inductance=1e-3  SetiL0=off  InitialCurrent=0  Capacitance=(Ccs1/2)*Len35_batt1_HVJB1_pos  Setx0=off  InitialVoltage=0  Measurements=None
  Series RLC Branch3 : spsSeriesRLCBranchLib/Series RLC Branch  LConnTagsString=__new0  RConnTagsString=__new0  BranchType=C  Resistance=1  Inductance=1e-3  SetiL0=off  InitialCurrent=0  Capacitance=(Ccs2/2)*Len35_batt1_HVJB1_neg  Setx0=off  InitialVoltage=0  Measurements=None
  Shield+ : spsSeriesRLCBranchLib/Series RLC Branch  LConnTagsString=__new0  RConnTagsString=__new0  BranchType=R  Resistance=Rs1*Len35_batt1_HVJB1_pos  Inductance=Lps95*3.270  SetiL0=off  InitialCurrent=0  Capacitance=1e-6  Setx0=off  InitialVoltage=0  Measurements=Branch voltage and current
  Shield- : spsSeriesRLCBranchLib/Series RLC Branch  LConnTagsString=__new0  RConnTagsString=__new0  BranchType=R  Resistance=Rs2*Len35_batt1_HVJB1_neg  Inductance=Lns95*3.305  SetiL0=off  InitialCurrent=0  Capacitance=1e-6  Setx0=off  InitialVoltage=0  Measurements=Branch voltage and current
  +Ve IN : PMIOPort  Side=Left
  -Ve OUT : PMIOPort  Port=2  Side=Left
  +Ve OUT : PMIOPort  Port=3  Side=Right
  -Ve IN : PMIOPort  Port=4  Side=Right
  connections:
  Series RLC Branch3/LConn1 -- -Ve OUT/RConn1 -- Core-/LConn1
  Ground/LConn1 -- Rg/RConn1
  Series RLC Branch2/LConn1 -- +Ve IN/RConn1 -- Core+/LConn1
  Series RLC Branch/LConn1 -- +Ve OUT/RConn1 -- Core+/RConn1
  Series RLC Branch/RConn1 -- Shield+/RConn1 -- Series RLC Branch1/RConn1 -- Shield-/RConn1 -- Series RLC Branch3/RConn1 -- Shield-/LConn1 -- Shield+/LConn1 -- Series RLC Branch2/RConn1 -- Rg/LConn1
  -Ve IN/RConn1 -- Series RLC Branch1/LConn1 -- Core-/RConn1

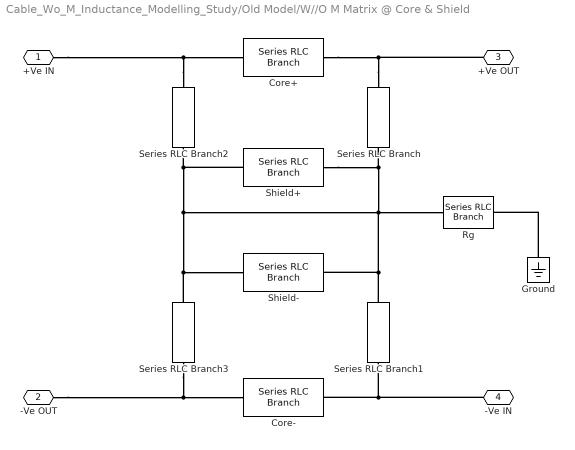
== system Cable_Wo_M_Inductance_Modelling_Study/Old Model/W//O M Matrix @ Core & Shield ==
  Core+ : spsSeriesRLCBranchLib/Series RLC Branch  LConnTagsString=__new0  RConnTagsString=__new0  BranchType=RL  Resistance=Rc1*Len35_batt1_HVJB1_pos  Inductance=Lc1_total*Len35_batt1_HVJB1_pos  SetiL0=off  InitialCurrent=0  Capacitance=1e-6  Setx0=off  InitialVoltage=0  Measurements=Branch voltage and current
  Core- : spsSeriesRLCBranchLib/Series RLC Branch  LConnTagsString=__new0  RConnTagsString=__new0  BranchType=RL  Resistance=Rc2*Len35_batt1_HVJB1_neg  Inductance=Lc2_total*Len35_batt1_HVJB1_neg  SetiL0=off  InitialCurrent=0  Capacitance=1e-6  Setx0=off  InitialVoltage=0  Measurements=Branch voltage and current
  Ground : spsGroundLib/Ground  LConnTagsString=a
  Rg : spsSeriesRLCBranchLib/Series RLC Branch  LConnTagsString=__new0  RConnTagsString=__new0  BranchType=R  Resistance=10e-03  Inductance=1e-3  SetiL0=off  InitialCurrent=0  Capacitance=1e-6  Setx0=off  InitialVoltage=0  Measurements=Branch voltage and current
  Series RLC Branch : spsSeriesRLCBranchLib/Series RLC Branch  LConnTagsString=__new0  RConnTagsString=__new0  BranchType=C  Resistance=1  Inductance=1e-3  SetiL0=off  InitialCurrent=0  Capacitance=(Ccs1/2)*Len35_batt1_HVJB1_pos  Setx0=off  InitialVoltage=0  Measurements=None
  Series RLC Branch1 : spsSeriesRLCBranchLib/Series RLC Branch  LConnTagsString=__new0  RConnTagsString=__new0  BranchType=C  Resistance=1  Inductance=1e-3  SetiL0=off  InitialCurrent=0  Capacitance=(Ccs2/2)*Len35_batt1_HVJB1_neg  Setx0=off  InitialVoltage=0  Measurements=None
  Series RLC Branch2 : spsSeriesRLCBranchLib/Series RLC Branch  LConnTagsString=__new0  RConnTagsString=__new0  BranchType=C  Resistance=1  Inductance=1e-3  SetiL0=off  InitialCurrent=0  Capacitance=(Ccs1/2)*Len35_batt1_HVJB1_pos  Setx0=off  InitialVoltage=0  Measurements=None
  Series RLC Branch3 : spsSeriesRLCBranchLib/Series RLC Branch  LConnTagsString=__new0  RConnTagsString=__new0  BranchType=C  Resistance=1  Inductance=1e-3  SetiL0=off  InitialCurrent=0  Capacitance=(Ccs2/2)*Len35_batt1_HVJB1_neg  Setx0=off  InitialVoltage=0  Measurements=None
  Shield+ : spsSeriesRLCBranchLib/Series RLC Branch  LConnTagsString=__new0  RConnTagsString=__new0  BranchType=RL  Resistance=Rs1*Len35_batt1_HVJB1_pos  Inductance=Ls1_eff*Len35_batt1_HVJB1_pos  SetiL0=off  InitialCurrent=0  Capacitance=1e-6  Setx0=off  InitialVoltage=0  Measurements=Branch voltage and current
  Shield- : spsSeriesRLCBranchLib/Series RLC Branch  LConnTagsString=__new0  RConnTagsString=__new0  BranchType=RL  Resistance=Rs2*Len35_batt1_HVJB1_neg  Inductance=Ls2_eff*Len35_batt1_HVJB1_neg  SetiL0=off  InitialCurrent=0  Capacitance=1e-6  Setx0=off  InitialVoltage=0  Measurements=Branch voltage and current
  +Ve IN : PMIOPort  Side=Left
  -Ve OUT : PMIOPort  Port=2  Side=Left
  +Ve OUT : PMIOPort  Port=3  Side=Right
  -Ve IN : PMIOPort  Port=4  Side=Right
  connections:
  Series RLC Branch3/LConn1 -- -Ve OUT/RConn1 -- Core-/LConn1
  Ground/LConn1 -- Rg/RConn1
  Series RLC Branch2/LConn1 -- +Ve IN/RConn1 -- Core+/LConn1
  Series RLC Branch/LConn1 -- +Ve OUT/RConn1 -- Core+/RConn1
  Series RLC Branch/RConn1 -- Shield+/RConn1 -- Series RLC Branch1/RConn1 -- Shield-/RConn1 -- Series RLC Branch3/RConn1 -- Shield-/LConn1 -- Shield+/LConn1 -- Series RLC Branch2/RConn1 -- Rg/LConn1
  -Ve IN/RConn1 -- Series RLC Branch1/LConn1 -- Core-/RConn1
